simulink model "Wind_PMSG_Transient_R3"  (R2026a)
settings: Solver=ode15s  StopTime=Base.Simulation.StopTime  MaxStep=Base.Simulation.MaxStep
InitFcn:
  | root=fileparts(fileparts(get_param(bdroot,'FileName'))); run(fullfile(root,'parameters','init_wind_pmsg_transient_r3.m'));
undefined symbols (not defined in the file): Base, Control, Converter, Drive, Filter, Grid, PMSG, Wind
libraries: nesl_utility x14, ee_lib x12, fl_lib x4, simulink x2
(part 1 of 2)
Description:
  | Derived transient model: two-mass direct-drive shaft, explicit PMSG dq states and average MSC FOC feeding the accepted switching GSC and grid interface.
settings Model: Creator=fakebob2004  LastModifiedBy=fakebob2004

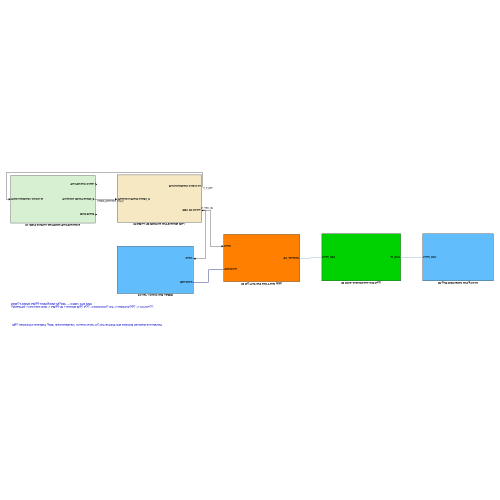
[thumbnail: Simulink's stored preview of the top-level diagram]
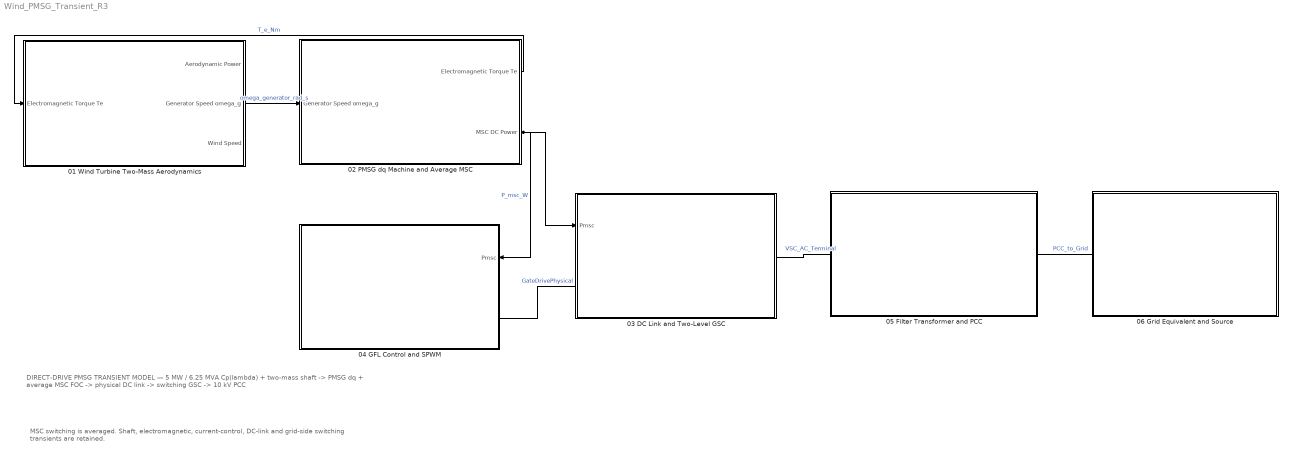
== system Wind_PMSG_Transient_R3 ==
  note: DIRECT-DRIVE PMSG TRANSIENT MODEL — 5 MW / 6.25 MVA
      | Cp(lambda) + two-mass shaft -> PMSG dq + average MSC FOC -> physical DC link -> switching GSC -> 10 kV PCC
  note: MSC switching is averaged. Shaft, electromagnetic, current-control, DC-link and grid-side switching transients are retained.
  01 Wind Turbine Two-Mass Aerodynamics : Subsystem
  02 PMSG dq Machine and Average MSC : Subsystem
  03 DC Link and Two-Level GSC : Subsystem
  04 GFL Control and SPWM : Subsystem
      settings: PortSchema="{\"entries\":[{\"content\":{\"sides\":[{\"content\":{},\"type\":\"ConnectorPlacement.EquallySpacedRectSide\",\"uuid\":\"96295b0e-7f92-4eb5-94fb-1e379a07647e\"},{\"content\":{\"connectorIds\":[\"In1\",\"RConn1\"],\"side\":\"RIGHT\"},\"type\":\"ConnectorPlacement.EquallySpacedRectSide\",\"uuid\":\"831b7b8f-9668-4ddf-9feb-732f61fa57d8\"},{\"content\":{\"side\":\"TOP\"},\"type\":\"ConnectorPlacement.EquallySpacedRectSide\",\"uuid\":\"f19125e2-22e2-45e6-ab3f-ff5603225915\"},{\"content\":{\"side\":\"BOTTOM\"},\"type\":\"ConnectorPlacement.EquallySpacedRectSide\",\"uuid\":\"5342ef29-4f2f-4bd8-ad29-4f76b3f65d35\"}]},\"type\":\"ConnectorPlacement.EquallySpacedConnector\",\"uuid\":\"9af9a57b-5404-446b-bd5e-01cd06fadf4a\"}],\"packageUris\":[\"http://schema.mathworks.com/mf0/Connector/R2020b\"],\"version\":\"1.0\"}"
  05 Filter Transformer and PCC : Subsystem
  06 Grid Equivalent and Source : Subsystem
  wires:
  01 Wind Turbine Two-Mass Aerodynamics/2(Generator Speed omega_g) -> 02 PMSG dq Machine and Average MSC/1(Generator Speed omega_g)  "omega_generator_rad_s"
  02 PMSG dq Machine and Average MSC/1(Electromagnetic Torque Te) -> 01 Wind Turbine Two-Mass Aerodynamics/1(Electromagnetic Torque Te)  "T_e_Nm"
  02 PMSG dq Machine and Average MSC/2(MSC DC Power) -> 03 DC Link and Two-Level GSC/1(Pmsc), 04 GFL Control and SPWM/1(Pmsc)  "P_msc_W"
  connections:
  03 DC Link and Two-Level GSC/RConn1 -- 05 Filter Transformer and PCC/LConn1  "VSC_AC_Terminal"
  05 Filter Transformer and PCC/RConn1 -- 06 Grid Equivalent and Source/LConn1  "PCC_to_Grid"
  04 GFL Control and SPWM/RConn1 -- 03 DC Link and Two-Level GSC/LConn1  "GateDrivePhysical"

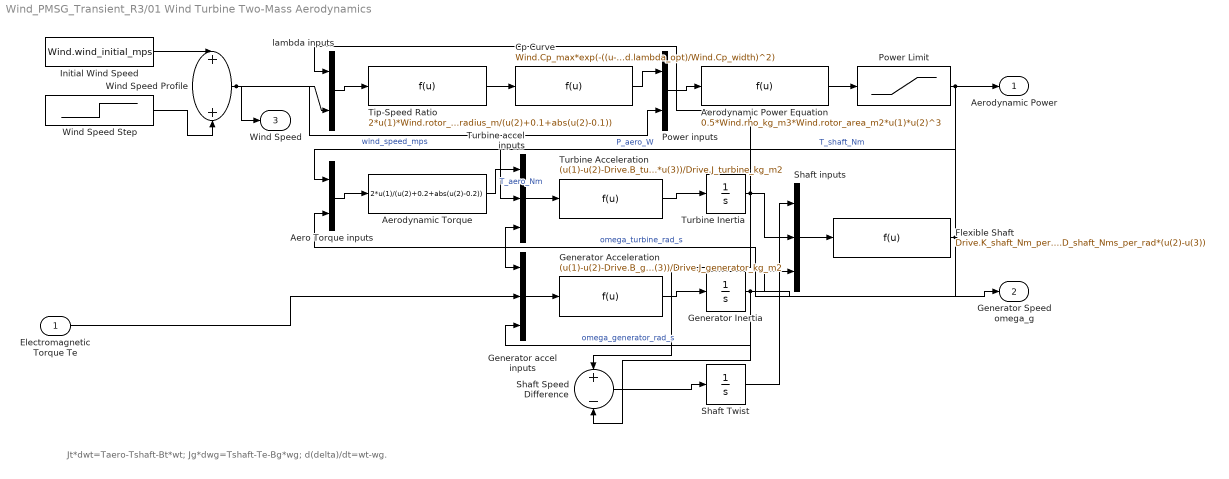
== system Wind_PMSG_Transient_R3/01 Wind Turbine Two-Mass Aerodynamics ==
  note: Jt*dwt=Taero-Tshaft-Bt*wt; Jg*dwg=Tshaft-Te-Bg*wg; d(delta)/dt=wt-wg.
  Electromagnetic Torque Te : Inport
  Aero Torque inputs : Mux  Inputs=2
  Aerodynamic Power Equation : Fcn  Expr=0.5*Wind.rho_kg_m3*Wind.rotor_area_m2*u(1)*u(2)^3
  Aerodynamic Torque : Fcn  Expr=2*u(1)/(u(2)+0.2+abs(u(2)-0.2))
  Cp Curve : Fcn  Expr=Wind.Cp_max*exp(-((u-Wind.lambda_opt)/Wind.Cp_width)^2)
  Flexible Shaft : Fcn  Expr=Drive.K_shaft_Nm_per_rad*u(1)+Drive.D_shaft_Nms_per_rad*(u(2)-u(3))
  Generator Acceleration : Fcn  Expr=(u(1)-u(2)-Drive.B_generator_Nms_per_rad*u(3))/Drive.J_generator_kg_m2
  Generator Inertia : Integrator  InitialCondition=PMSG.Init.omega_rad_s
  Generator accel inputs : Mux  Inputs=3
  Initial Wind Speed : Constant  Value=Wind.wind_initial_mps
  Power Limit : Saturate  UpperLimit=1.10*Wind.P_rated_W  LowerLimit=0
  Power inputs : Mux  Inputs=2
  Shaft Speed Difference : Sum  Inputs=+-
  Shaft Twist : Integrator  InitialCondition=PMSG.Init.shaft_angle_rad
  Shaft inputs : Mux  Inputs=3
  Tip-Speed Ratio : Fcn  Expr=2*u(1)*Wind.rotor_radius_m/(u(2)+0.1+abs(u(2)-0.1))
  Turbine Acceleration : Fcn  Expr=(u(1)-u(2)-Drive.B_turbine_Nms_per_rad*u(3))/Drive.J_turbine_kg_m2
  Turbine Inertia : Integrator  InitialCondition=PMSG.Init.omega_rad_s
  Turbine accel inputs : Mux  Inputs=3
  Wind Speed Profile : Sum
  Wind Speed Step : Step  Time=Wind.wind_step_time_s  FinalValue=Wind.wind_step_mps  SampleTime=0
  lambda inputs : Mux  Inputs=2
  Aerodynamic Power : Outport
  Generator Speed omega_g : Outport  Port=2
  Wind Speed : Outport  Port=3
  wires:
  Initial Wind Speed/1 -> Wind Speed Profile/1
  Wind Speed Step/1 -> Wind Speed Profile/2
  Wind Speed Profile/1 -> Wind Speed/1, lambda inputs/2, Power inputs/2  "wind_speed_mps"
  Turbine Inertia/1 -> lambda inputs/1, Aero Torque inputs/2, Turbine accel inputs/3, Shaft Speed Difference/1, Shaft inputs/2  "omega_turbine_rad_s"
  lambda inputs/1 -> Tip-Speed Ratio/1
  Tip-Speed Ratio/1 -> Cp Curve/1
  Cp Curve/1 -> Power inputs/1
  Power inputs/1 -> Aerodynamic Power Equation/1
  Aerodynamic Power Equation/1 -> Power Limit/1
  Power Limit/1 -> Aerodynamic Power/1, Aero Torque inputs/1  "P_aero_W"
  Aero Torque inputs/1 -> Aerodynamic Torque/1
  Aerodynamic Torque/1 -> Turbine accel inputs/1  "T_aero_Nm"
  Flexible Shaft/1 -> Turbine accel inputs/2, Generator accel inputs/1  "T_shaft_Nm"
  Turbine accel inputs/1 -> Turbine Acceleration/1
  Turbine Acceleration/1 -> Turbine Inertia/1
  Electromagnetic Torque Te/1 -> Generator accel inputs/2
  Generator Inertia/1 -> Generator accel inputs/3, Shaft Speed Difference/2, Shaft inputs/3, Generator Speed omega_g/1  "omega_generator_rad_s"
  Generator accel inputs/1 -> Generator Acceleration/1
  Generator Acceleration/1 -> Generator Inertia/1
  Shaft Speed Difference/1 -> Shaft Twist/1
  Shaft Twist/1 -> Shaft inputs/1
  Shaft inputs/1 -> Flexible Shaft/1

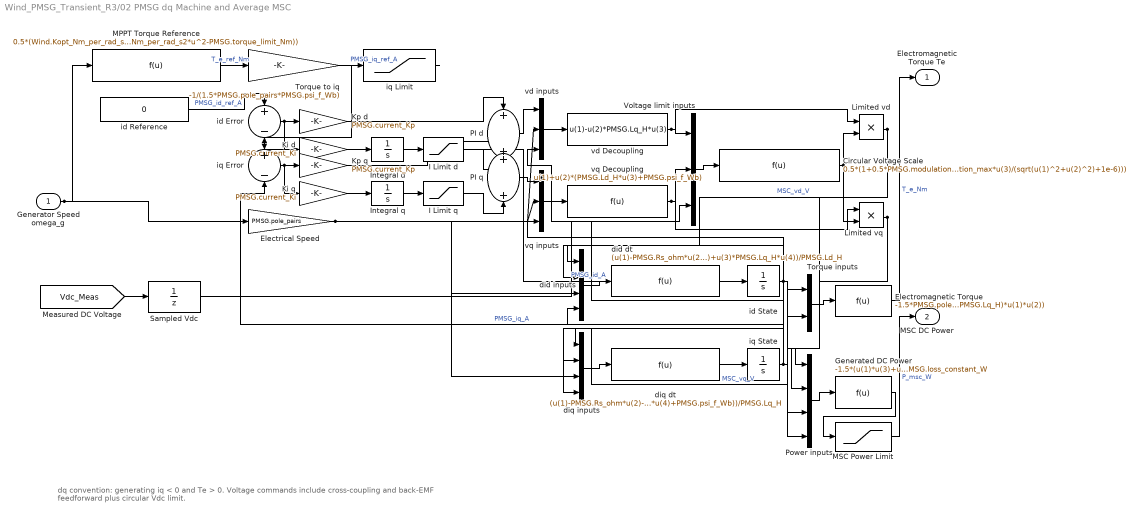
== system Wind_PMSG_Transient_R3/02 PMSG dq Machine and Average MSC ==
  note: dq convention: generating iq < 0 and Te > 0. Voltage commands include cross-coupling and back-EMF feedforward plus circular Vdc limit.
  Generator Speed omega_g : Inport
  Circular Voltage Scale : Fcn  Expr=0.5*(1+0.5*PMSG.modulation_max*u(3)/(sqrt(u(1)^2+u(2)^2)+1e-6)-abs(1-0.5*PMSG.modulation_max*u(3)/(sqrt(u(1)^2+u(2)^2)+1e-6)))
  Electrical Speed : Gain  Gain=PMSG.pole_pairs
  Electromagnetic Torque : Fcn  Expr=-1.5*PMSG.pole_pairs*(PMSG.psi_f_Wb*u(2)+(PMSG.Ld_H-PMSG.Lq_H)*u(1)*u(2))
  Generated DC Power : Fcn  Expr=-1.5*(u(1)*u(3)+u(2)*u(4))*PMSG.msc_efficiency-PMSG.loss_constant_W
  I Limit d : Saturate  UpperLimit=PMSG.integrator_limit_V  LowerLimit=-PMSG.integrator_limit_V
  I Limit q : Saturate  UpperLimit=PMSG.integrator_limit_V  LowerLimit=-PMSG.integrator_limit_V
  Integral d : Integrator  InitialCondition=PMSG.Init.vd_pi_V
  Integral q : Integrator  InitialCondition=PMSG.Init.vq_pi_V
  Ki d : Gain  Gain=PMSG.current_Ki
  Ki q : Gain  Gain=PMSG.current_Ki
  Kp d : Gain  Gain=PMSG.current_Kp
  Kp q : Gain  Gain=PMSG.current_Kp
  Limited vd : Product
  Limited vq : Product
  MPPT Torque Reference : Fcn  Expr=0.5*(Wind.Kopt_Nm_per_rad_s2*u^2+PMSG.torque_limit_Nm-abs(Wind.Kopt_Nm_per_rad_s2*u^2-PMSG.torque_limit_Nm))
  MSC Power Limit : Saturate  UpperLimit=PMSG.Sn_W  LowerLimit=0
  PI d : Sum
  PI q : Sum
  Power inputs : Mux
  Sampled Vdc : UnitDelay  InitialCondition=Converter.Vdc_nom  SampleTime=Control.Ts
  Torque inputs : Mux  Inputs=2
  Torque to iq : Gain  Gain=-1/(1.5*PMSG.pole_pairs*PMSG.psi_f_Wb)
  Voltage limit inputs : Mux  Inputs=3
  did dt : Fcn  Expr=(u(1)-PMSG.Rs_ohm*u(2)+u(3)*PMSG.Lq_H*u(4))/PMSG.Ld_H
  did inputs : Mux
  diq dt : Fcn  Expr=(u(1)-PMSG.Rs_ohm*u(2)-u(3)*(PMSG.Ld_H*u(4)+PMSG.psi_f_Wb))/PMSG.Lq_H
  diq inputs : Mux
  id Error : Sum  Inputs=+-
  id Reference : Constant  Value=0
  id State : Integrator  InitialCondition=PMSG.Init.id_A
  iq Error : Sum  Inputs=+-
  iq Limit : Saturate  UpperLimit=PMSG.current_limit_A  LowerLimit=-PMSG.current_limit_A
  iq State : Integrator  InitialCondition=PMSG.Init.iq_A
  vd Decoupling : Fcn  Expr=u(1)-u(2)*PMSG.Lq_H*u(3)
  vd inputs : Mux  Inputs=3
  vq Decoupling : Fcn  Expr=u(1)+u(2)*(PMSG.Ld_H*u(3)+PMSG.psi_f_Wb)
  vq inputs : Mux  Inputs=3
  Electromagnetic Torque Te : Outport
  MSC DC Power : Outport  Port=2
  wires:
  Generator Speed omega_g/1 -> MPPT Torque Reference/1, Electrical Speed/1
  MPPT Torque Reference/1 -> Torque to iq/1  "T_e_ref_Nm"
  Torque to iq/1 -> iq Limit/1
  iq Limit/1 -> iq Error/1  "PMSG_iq_ref_A"
  id Reference/1 -> id Error/1  "PMSG_id_ref_A"
  id State/1 -> id Error/2, vq inputs/3, did inputs/2, diq inputs/4, Torque inputs/1, Power inputs/3  "PMSG_id_A"
  iq State/1 -> iq Error/2, vd inputs/3, did inputs/4, diq inputs/2, Torque inputs/2, Power inputs/4  "PMSG_iq_A"
  id Error/1 -> Kp d/1, Ki d/1
  Ki d/1 -> Integral d/1
  Integral d/1 -> I Limit d/1
  Kp d/1 -> PI d/1
  I Limit d/1 -> PI d/2
  iq Error/1 -> Kp q/1, Ki q/1
  Ki q/1 -> Integral q/1
  Integral q/1 -> I Limit q/1
  Kp q/1 -> PI q/1
  I Limit q/1 -> PI q/2
  PI d/1 -> vd inputs/1
  Electrical Speed/1 -> vd inputs/2, vq inputs/2, did inputs/3, diq inputs/3
  vd inputs/1 -> vd Decoupling/1
  PI q/1 -> vq inputs/1
  vq inputs/1 -> vq Decoupling/1
  vd Decoupling/1 -> Voltage limit inputs/1, Limited vd/1
  vq Decoupling/1 -> Voltage limit inputs/2, Limited vq/1
  [Vdc_Meas] -> Sampled Vdc/1
  Sampled Vdc/1 -> Voltage limit inputs/3
  Voltage limit inputs/1 -> Circular Voltage Scale/1
  Circular Voltage Scale/1 -> Limited vd/2, Limited vq/2
  Limited vd/1 -> did inputs/1, Power inputs/1  "MSC_vd_V"
  did inputs/1 -> did dt/1
  did dt/1 -> id State/1
  Limited vq/1 -> diq inputs/1, Power inputs/2  "MSC_vq_V"
  diq inputs/1 -> diq dt/1
  diq dt/1 -> iq State/1
  Torque inputs/1 -> Electromagnetic Torque/1
  Electromagnetic Torque/1 -> Electromagnetic Torque Te/1  "T_e_Nm"
  Power inputs/1 -> Generated DC Power/1
  Generated DC Power/1 -> MSC Power Limit/1
  MSC Power Limit/1 -> MSC DC Power/1  "P_msc_W"

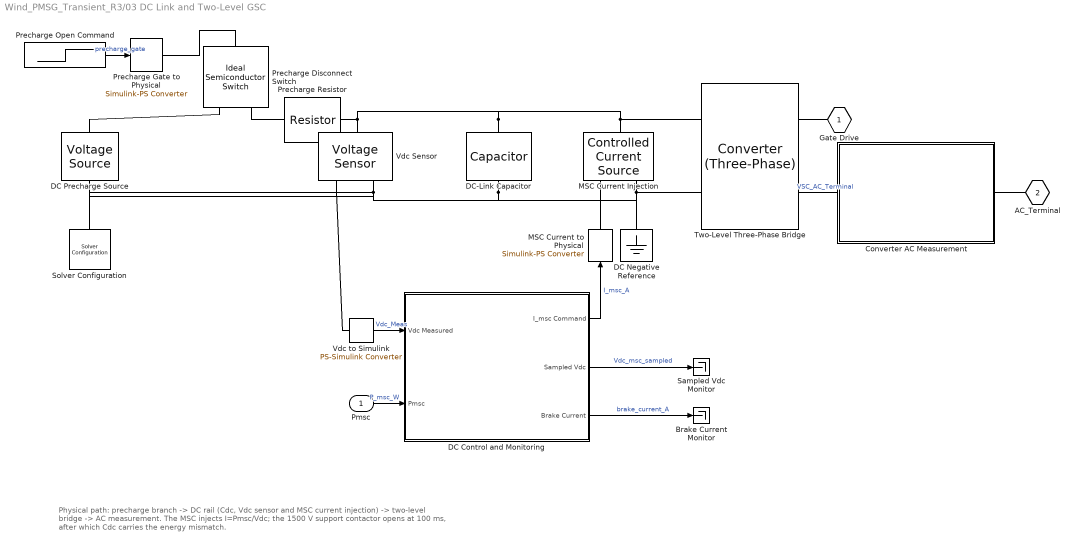
== system Wind_PMSG_Transient_R3/03 DC Link and Two-Level GSC ==
  note: Physical path: precharge branch -> DC rail (Cdc, Vdc sensor and MSC current injection) -> two-level bridge -> AC measurement.
      | The MSC injects I=Pmsc/Vdc; the 1500 V support contactor opens at 100 ms, after which Cdc carries the energy mismatch.
  Pmsc : Inport
  Brake Current Monitor : Terminator
  Converter AC Measurement : Subsystem
  DC Control and Monitoring : Subsystem
  DC Negative Reference : fl_lib/Electrical/Electrical Elements/Electrical Reference
  DC Precharge Source : ee_lib/Sources/Voltage Source  dc_voltage=Converter.Vdc_nom V  ac_voltage=0 V  ac_shift=0 rad  ac_frequency=60 Hz  noise_mode=ee.enum.sources.noise.Disabled  PSD=0 V^2/Hz  sample_time=1e-3 s  repeatability=ee.enum.sources.repeatability.NotRepeatable  user_seed=0  auto_seed=3499211588  i_specify=off  i_priority=None  i=0 A  i_nominal_specify=off  i_nominal_value=1  i_nominal_unit=A  v_specify=off  v_priority=None  v=0 V  v_nominal_specify=off  v_nominal_value=1  v_nominal_unit=V
  DC-Link Capacitor : ee_lib/Passive/Capacitor  cap_option=ee.enum.passive.capacitor.capOption.const  c=Converter.Cdc F  Cvec=[1e-05, 1e-06] F  Vvec=[0, 10] V  CV_table_symmetry=ee.enum.passive.capacitor.tableSymmetry.yes  f_vec=[1, 10] kHz  DFext_vec=[.8, 1.2]  enable_C_tol=ee.enum.toleranceApplication.none  averaging_period=0 s  C_tol=5  tol_distribution=ee.enum.toleranceDistribution.uniform  nSigma=4  r=Converter.Cdc_esr Ohm  g=0 1/Ohm  enable_operating_limits=ee.enum.enable.no  operating_limit_action=ee.enum.passive.reportOpLim.warn  max_working_voltage_range=[-25, 25] V  power_rating=1 W  maxTemperature=85 degC  thermalEnable=false  thermalMass=1 J/K  i_specify=off  i_priority=None  i=0 A  i_nominal_specify=off  i_nominal_value=1  i_nominal_unit=A  v_specify=on  v_priority=High  v=Converter.Vdc_nom V  v_nominal_specify=off  v_nominal_value=1  v_nominal_unit=V  vc_specify=off  vc_priority=High  vc=0 V  vc_nominal_specify=off  vc_nominal_value=1  vc_nominal_unit=V  T_specify=off  T_priority=None  T=298.15 K  T_nominal_specify=off  T_nominal_value=1  T_nominal_unit=K
  MSC Current Injection : fl_lib/Electrical/Electrical Sources/Controlled Current Source
  MSC Current to Physical : nesl_utility/Simulink-PS Converter  PhysicalDomain=network_engine_domain  SubClassName=ps_input  LeftPortType=input  RightPortType=output  PseudoPeriodic=off  Frequencies=[]  NoiseDistribution=none  NoiseParameters=[]  Unit=A  AffineConversion=off  FilteringAndDerivatives=provide  SimscapeFilterOrder=1  InputFilterTimeConstant=0.001  UdotUserProvided=0
  Precharge Disconnect Switch : ee_lib/Semiconductors & Converters/Ideal Semiconductor Switch  port_option=ee.enum.controlport.ps  Ron=Wind.brake_switch_Ron_ohm Ohm  Goff=Wind.brake_switch_Goff_S 1/Ohm  Vth=0.5 V  diode_param=ee.enum.semiconductors.protectionDiode.external  diode_Vf=0.8 V  diode_Ron=0.001 Ohm  diode_Goff=1e-5 1/Ohm  diode_C=50e-9 F  diode_iRM=-235 A  diode_iF=300 A  diode_idot=-50 A/us  diode_trr_param=ee.enum.converters.diodetrr.trr_factor  diode_trr_factor=3  diode_trr=15 us  diode_Qrr=1500 s*uA
  Precharge Gate to Physical : nesl_utility/Simulink-PS Converter  PhysicalDomain=network_engine_domain  SubClassName=ps_input  LeftPortType=input  RightPortType=output  PseudoPeriodic=off  Frequencies=[]  NoiseDistribution=none  NoiseParameters=[]  Unit=1  AffineConversion=off  FilteringAndDerivatives=provide  SimscapeFilterOrder=1  InputFilterTimeConstant=0.001  UdotUserProvided=0
  Precharge Open Command : Step  Time=Wind.precharge_open_time_s  InitialValue=1  FinalValue=0  SampleTime=0
  Precharge Resistor : ee_lib/Passive/Resistor  R=Wind.precharge_R_ohm Ohm  enable_R_tol=ee.enum.toleranceApplication.none  R_tol=5  tol_distribution=ee.enum.toleranceDistribution.uniform  nSigma=4  enable_operating_limits=ee.enum.enable.no  operating_limit_action=ee.enum.passive.reportOpLim.warn  power_rating=1 W  max_working_voltage=100 V  noise_mode=ee.enum.sources.noise.Disabled  Tdevice=25 degC  sample_time=1e-3 s  repeatability=ee.enum.ic.repeatability.notRepeatable  user_seed=0  auto_seed=3890346746  power_derating_T1=70 degC  power_derating_T2=155 degC  operating_temperature_range_vec=[-50, 150] degC  alpha=3.93e-3 1/K  Tmeas=25 degC  thermal_mass=100 J/K  temperature_specify=off  temperature_priority=High  temperature=298.15 K  temperature_nominal_specify=off  temperature_nominal_value=1  temperature_nominal_unit=K
  Sampled Vdc Monitor : Terminator
  Solver Configuration : nesl_utility/Solver Configuration  PhysicalDomain=network_engine_domain  SubClassName=solver  LeftPortType=input  RightPortType=generic  Tones=[]  Harmonics=[]  SimulateNoise=off  Profile=off  UseLocalSampling=off  EnableSwitchedLinearOptims=on  FrequencyDomain=off  UseCCode=off  RelTol=0.001  AbsTol=0.001  MinStep=1e-09  ToWorkspace=off  RevertToSquareIcSolve=off  NumHomotopyIterations=100  PhasorMode=off  PhasorModeNumHarmonics=1  ConsistencySolver=NEWTON_XTOL_AFTER_FTOL  CanonicalOrdering=CANONICAL  OptimizeIntermediates=OPTIMIZED  IndexReductionMethod=DerivativeReplacement  DoDC=off  ResidualTolerance=1e-09  ConsistencyTolSource=GLOBAL  ConsistencyAbsTol=0.001  ConsistencyRelTol=0.001  ConsistencyTolFactor=0.001  UseLocalSolver=off  LocalSolverChoice=NE_BACKWARD_EULER_ADVANCER  ResolveIndetEquations=on  FunctionEvalNumThread=1  LocalSolverSampleTime=0.001  DoFixedCost=off  MaxNonlinIter=3  MaxModeIter=2  ComputeImpulses=off  ImpulseIterations=2  LinearAlgebra=auto  LinearAlgebraNumThread=0  EquationFormulation=NE_TIME_EF  DelaysMemoryBudget=1024  AutomaticFiltering=on  FilteringTimeConstant=0.001  PartitionStorageMethod=AS_NEEDED  PartitionMemoryBudget=1024  PartitionMethod=ROBUST  MultibodyUseLocalSolver=off  MultibodyLocalSolverChoice=ODE1  MultibodyLocalSolverSampleTime=0.001
  Two-Level Three-Phase Bridge : ee_lib/Semiconductors & Converters/Converters/Converter (Three-Phase)  port_option=ee.enum.threePhasePort.composite  fidelity_option=ee.enum.converters.fidelity.detailed  device_type=ee.enum.converters.switchingdevice.ideal  showThermalPort=false  K=0  Vth=Converter.GateThresholdVoltage V  Vgt=1 V  Vgt_off=-1 V  Ih=1 A  Vf=0.8 V  Ron=Converter.SwitchOnResistance Ohm  Rds=0.001 Ohm  Goff=Converter.OffConductance 1/Ohm  Eon_scalar=22.86e-3 J  Eoff_scalar=17.14e-3 J  Eoff_natural_commutation=10e-3 J  Voff=300 V  Iout_scalar=600 A  onCurrentMeasDelay=0 s  useCurrentFromPreviousCycle=false  useVoltageFromPreviousCycle=false  diode_param=ee.enum.converters.protectiondiode.nodynamics  diode_Vf=0.8 V  diode_Ron=0.001 Ohm  diode_Goff=1e-5 1/Ohm  diode_C=50 nF  diode_iRM=-235 A  diode_iF=300 A  diode_idot=-50 A/us  diode_trr_param=ee.enum.converters.diodetrr.trr_factor  diode_trr_factor=3  diode_trr=15 us  diode_Qrr=1500 s*uA  diode_rec_loss_model=ee.enum.diode.reverseRecoveryModel.fixed  diode_ErecVal=0 J  diode_scaleWithIandV=false  diode_ErecMat=zeros(2, 3) J  diode_TjrecVec=[298.15, 398.15] K  diode_IfrecVec=[.1, 1, 10] A  diode_IrecVal=10 A  diode_VrecVal=10 V  diode_tFilter=1 / 1000 / 100 s  thermal_network_parameterization=ee.enum.thermalNetworkTopology.external  Rth=[.08, .5] K/W  Rth_Cauer=[.08, .1, .5] K/W  Rth_Foster=[.08, .14, .22, .16] K/W  thermal_mass_parameterization=ee.enum.thermalNetwork.timeconstant  thermal_mass=[.01, .5] J/K  thermal_mass_Cauer=[.01, .1, .5] J/K  thermal_mass_Foster=[.001, .005, .05, .5] J/K  thermal_time_constant=[.001, .2] s  thermal_time_constant_Cauer=[.001, .1, .2] s  thermal_time_constant_Foster=[7e-05, .0007, .01, .08] s  thermal_mass_initial_temperatures=[25, 25] degC  thermal_mass_initial_temperatures_Cauer=[25, 25, 25] degC  junction_thermal_mass=0.01 J/K  Tvec_initial_Foster=[25, 25, 25, 25] degC  snubber_type=ee.enum.converters.snubber.exclude  Cs=1e-7 F  Rs=0.1 Ohm  Vce_loss=[0, 150, 300] V
  Vdc Sensor : fl_lib/Electrical/Electrical Sensors/Voltage Sensor
  Vdc to Simulink : nesl_utility/PS-Simulink Converter  PhysicalDomain=network_engine_domain  SubClassName=ps_output  LeftPortType=input  RightPortType=output  PseudoPeriodic=off  Frequencies=[]  VectorFormat=inherit  Unit=V  AffineConversion=off
  Gate Drive : PMIOPort  Side=Left
  AC_Terminal : PMIOPort  Port=2  Side=Right
  wires:
  Vdc to Simulink/1 -> DC Control and Monitoring/1(Vdc Measured)  "Vdc_Meas"
  Pmsc/1 -> DC Control and Monitoring/2(Pmsc)  "P_msc_W"
  DC Control and Monitoring/1(I_msc Command) -> MSC Current to Physical/1  "I_msc_A"
  DC Control and Monitoring/2(Sampled Vdc) -> Sampled Vdc Monitor/1  "Vdc_msc_sampled"
  DC Control and Monitoring/3(Brake Current) -> Brake Current Monitor/1  "brake_current_A"
  Precharge Open Command/1 -> Precharge Gate to Physical/1  "precharge_gate"
  connections:
  Gate Drive/RConn1 -- Two-Level Three-Phase Bridge/LConn1
  Vdc Sensor/RConn1 -- Vdc to Simulink/LConn1
  Two-Level Three-Phase Bridge/LConn2 -- Converter AC Measurement/LConn1  "VSC_AC_Terminal"
  Converter AC Measurement/RConn1 -- AC_Terminal/RConn1
  MSC Current to Physical/RConn1 -- MSC Current Injection/RConn1
  DC Precharge Source/LConn1 -- Precharge Disconnect Switch/RConn1
  Precharge Disconnect Switch/RConn2 -- Precharge Resistor/LConn1
  Vdc Sensor/LConn1 -- Precharge Resistor/RConn1 -- DC-Link Capacitor/LConn1 -- MSC Current Injection/LConn1 -- Two-Level Three-Phase Bridge/RConn1
  Vdc Sensor/RConn2 -- DC Precharge Source/RConn1 -- Solver Configuration/RConn1 -- DC-Link Capacitor/RConn1 -- Two-Level Three-Phase Bridge/RConn2 -- MSC Current Injection/RConn2 -- DC Negative Reference/LConn1
  Precharge Gate to Physical/RConn1 -- Precharge Disconnect Switch/LConn1

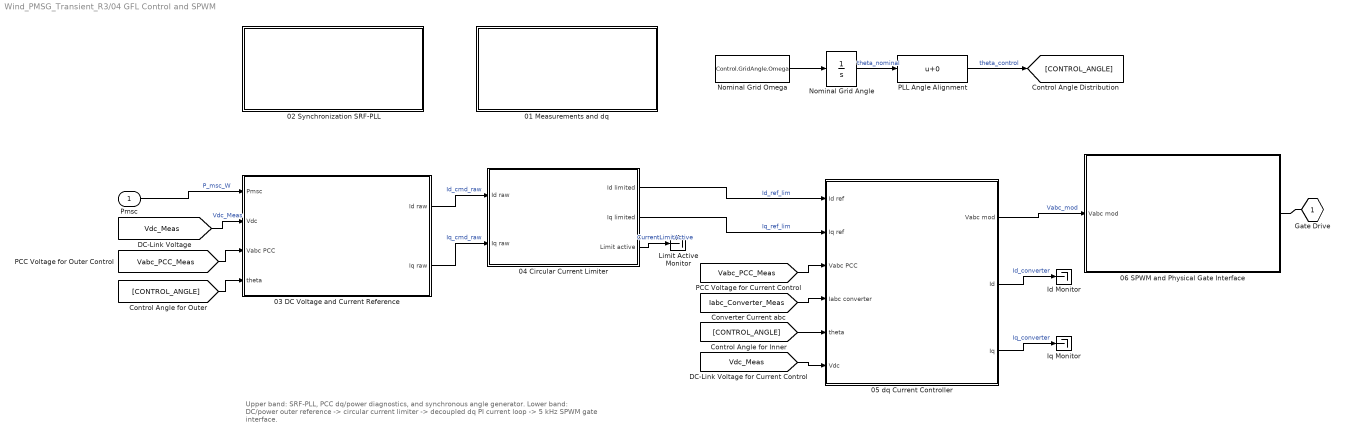
== system Wind_PMSG_Transient_R3/04 GFL Control and SPWM ==
  note: Upper band: SRF-PLL, PCC dq/power diagnostics, and synchronous angle generator. Lower band: DC/power outer reference -> circular current limiter -> decoupled dq PI current loop -> 5 kHz SPWM gate interface.
  Pmsc : Inport
  01 Measurements and dq : Subsystem
  02 Synchronization SRF-PLL : Subsystem
  03 DC Voltage and Current Reference : Subsystem
  04 Circular Current Limiter : Subsystem
  05 dq Current Controller : Subsystem
  06 SPWM and Physical Gate Interface : Subsystem
  Id Monitor : Terminator
  Iq Monitor : Terminator
  Limit Active Monitor : Terminator
  Nominal Grid Angle : Integrator  InitialCondition=Control.GridAngle.Theta0
  Nominal Grid Omega : Constant  Value=Control.GridAngle.Omega
  PLL Angle Alignment : Bias  SaturateOnIntegerOverflow=off
  Gate Drive : PMIOPort  Side=Right
  wires:
  Pmsc/1 -> 03 DC Voltage and Current Reference/1(Pmsc)  "P_msc_W"
  [Vdc_Meas] -> 03 DC Voltage and Current Reference/2(Vdc)  "Vdc_Meas"
  [Vabc_PCC_Meas] -> 03 DC Voltage and Current Reference/3(Vabc PCC)
  Nominal Grid Omega/1 -> Nominal Grid Angle/1
  Nominal Grid Angle/1 -> PLL Angle Alignment/1  "theta_nominal"
  PLL Angle Alignment/1 -> [CONTROL_ANGLE]  "theta_control"
  [CONTROL_ANGLE] -> 03 DC Voltage and Current Reference/4(theta)
  03 DC Voltage and Current Reference/1(Id raw) -> 04 Circular Current Limiter/1(Id raw)  "Id_cmd_raw"
  03 DC Voltage and Current Reference/2(Iq raw) -> 04 Circular Current Limiter/2(Iq raw)  "Iq_cmd_raw"
  04 Circular Current Limiter/1(Id limited) -> 05 dq Current Controller/1(Id ref)  "Id_ref_lim"
  04 Circular Current Limiter/2(Iq limited) -> 05 dq Current Controller/2(Iq ref)  "Iq_ref_lim"
  [Vabc_PCC_Meas] -> 05 dq Current Controller/3(Vabc PCC)
  [Iabc_Converter_Meas] -> 05 dq Current Controller/4(Iabc converter)
  [CONTROL_ANGLE] -> 05 dq Current Controller/5(theta)
  [Vdc_Meas] -> 05 dq Current Controller/6(Vdc)
  05 dq Current Controller/1(Vabc mod) -> 06 SPWM and Physical Gate Interface/1(Vabc mod)  "Vabc_mod"
  05 dq Current Controller/2(Id) -> Id Monitor/1  "Id_converter"
  05 dq Current Controller/3(Iq) -> Iq Monitor/1  "Iq_converter"
  04 Circular Current Limiter/3(Limit active) -> Limit Active Monitor/1  "CurrentLimitActive"
  connections:
  06 SPWM and Physical Gate Interface/RConn1 -- Gate Drive/RConn1

== system Wind_PMSG_Transient_R3/05 Filter Transformer and PCC ==
  note: Direct power path: Rf + Lf -> 0.69/10 kV Y-Y transformer -> PCC VI sensor. Measurements remain internal and logged.
  0.69 kV to 10 kV Step-Up Transformer : ee_lib/Passive/Transformers/Two-Winding Transformer (Three-Phase)  SRated=Transformer.Sn A*V  FRated=Transformer.f Hz  Winding1Connection=ee.enum.windingconnection.Y  VRated1=Transformer.Vll_primary V  Winding2Connection=ee.enum.windingconnection.Y  VRated2=Transformer.Vll_secondary V  CoreType=ee.enum.coretype.threelimb  pu_Rw1=Transformer.R1_pu  pu_Rw2=Transformer.R2_pu  leakage_reactance_option=ee.enum.transformer_leakage.exclude  pu_Xl1=Transformer.X1_pu  pu_Xl2=Transformer.X2_pu  magnetizing_resistance_option=ee.enum.transformer_magnetizingResistance.exclude  pu_Rm=500  magnetizing_reactance_option=ee.enum.transformer_magnetizingReactance.exclude  saturation_option=ee.enum.transformer_saturation.exclude  pu_Xm=Transformer.Xm_pu  current_data=[0, .002, 1, 2]  magnetic_flux_data=[0, 1.2, 1.5, 1.51]  pu_X0=0.5  i1_specify=off  i1_priority=None  i1=[0, 0, 0] A  i1_nominal_specify=off  i1_nominal_value=1  i1_nominal_unit=A  i2_specify=off  i2_priority=None  i2=[0, 0, 0] A  i2_nominal_specify=off  i2_nominal_value=1  i2_nominal_unit=A  phi_specify=off  phi_priority=None  phi=[0, 0, 0]  phi_nominal_specify=off  phi_nominal_value=1  phi_nominal_unit=1
  AC Filter Rf + Lf : ee_lib/Passive/RLC Assemblies/RLC (Three-Phase)  port_option=ee.enum.threePhasePort.composite  component_structure=ee.enum.rlc.structure.SeriesRL  R=Filter.R Ohm  L=Filter.L H  C=1e-6 F  R_parasitic=0 Ohm  G_parasitic=0 1/Ohm  IL_specify=off  IL_priority=High  IL=[0, 0, 0] A  IL_nominal_specify=off  IL_nominal_value=1  IL_nominal_unit=A  VC_specify=off  VC_priority=High  VC=[0, 0, 0] V  VC_nominal_specify=off  VC_nominal_value=1  VC_nominal_unit=V
  Iabc PCC to Simulink : nesl_utility/PS-Simulink Converter  PhysicalDomain=network_engine_domain  SubClassName=ps_output  LeftPortType=input  RightPortType=output  PseudoPeriodic=off  Frequencies=[]  VectorFormat=inherit  Unit=A  AffineConversion=off
  PCC VI Sensor : ee_lib/Sensors & Transducers/Current and Voltage Sensor (Three-Phase)  port_option=ee.enum.threePhasePort.composite  vMeasurementType=ee.enum.vmeasurement.lg  outputUnit=ee.enum.unit.si  SRated=Base.Sn A*V  VRated=Base.Vll_hv V  I_specify=off  I_priority=None  I=[0, 0, 0] A  I_nominal_specify=off  I_nominal_value=1  I_nominal_unit=A  V_specify=off  V_priority=None  V=[0, 0, 0] V  V_nominal_specify=off  V_nominal_value=1  V_nominal_unit=V
  Vabc PCC to Simulink : nesl_utility/PS-Simulink Converter  PhysicalDomain=network_engine_domain  SubClassName=ps_output  LeftPortType=input  RightPortType=output  PseudoPeriodic=off  Frequencies=[]  VectorFormat=inherit  Unit=V  AffineConversion=off
  From_VSC : PMIOPort  Side=Left
  To_Grid : PMIOPort  Port=2  Side=Right
  tag scope: Iabc_PCC_Meas=global, Vabc_PCC_Meas=global
  wires:
  Vabc PCC to Simulink/1 -> [Vabc_PCC_Meas]  "Vabc_PCC_Meas"
  Iabc PCC to Simulink/1 -> [Iabc_PCC_Meas]  "Iabc_PCC_Meas"
  connections:
  From_VSC/RConn1 -- AC Filter Rf + Lf/LConn1
  AC Filter Rf + Lf/RConn1 -- 0.69 kV to 10 kV Step-Up Transformer/LConn1
  0.69 kV to 10 kV Step-Up Transformer/RConn1 -- PCC VI Sensor/LConn1
  PCC VI Sensor/RConn3 -- To_Grid/RConn1
  PCC VI Sensor/RConn1 -- Vabc PCC to Simulink/LConn1
  PCC VI Sensor/RConn2 -- Iabc PCC to Simulink/LConn1

== system Wind_PMSG_Transient_R3/06 Grid Equivalent and Source ==
  note: Single Thevenin impedance: explicit SCR-based Rg + Lg followed by an ideal grounded-wye source (internal source impedance OFF).
  Grid Equivalent Rg + Lg : ee_lib/Passive/RLC Assemblies/RLC (Three-Phase)  port_option=ee.enum.threePhasePort.composite  component_structure=ee.enum.rlc.structure.SeriesRL  R=Grid.R Ohm  L=Grid.L H  C=1e-6 F  R_parasitic=0 Ohm  G_parasitic=0 1/Ohm  IL_specify=off  IL_priority=High  IL=[0, 0, 0] A  IL_nominal_specify=off  IL_nominal_value=1  IL_nominal_unit=A  VC_specify=off  VC_priority=High  VC=[0, 0, 0] V  VC_nominal_specify=off  VC_nominal_value=1  VC_nominal_unit=V
  Grid Neutral Ground : fl_lib/Electrical/Electrical Elements/Electrical Reference
  Ideal Three-Phase Grid Source : ee_lib/Sources/Voltage Source (Three-Phase)  vline_rms=Grid.Vll V  shift=Grid.phase_deg deg  freq=Grid.f Hz  impedance_option=0  SShortCircuit=1e6 A*V  XR=15  R=0.01 Ohm  L=3.97e-4 H  harmonic_option=0  harmonic_orders=[5, 7, 11, 13]  harmonic_ratios=[.1, .1, .1, .1]  G_parasitic=0 1/Ohm  I_specify=off  I_priority=None  I=[0, 0, 0] A  I_nominal_specify=off  I_nominal_value=1  I_nominal_unit=A
  From_PCC : PMIOPort  Side=Left
  connections:
  From_PCC/RConn1 -- Grid Equivalent Rg + Lg/LConn1
  Grid Equivalent Rg + Lg/RConn1 -- Ideal Three-Phase Grid Source/RConn1
  Ideal Three-Phase Grid Source/LConn1 -- Grid Neutral Ground/LConn1

== system Wind_PMSG_Transient_R3/03 DC Link and Two-Level GSC/Converter AC Measurement ==
  note: VSC-side phase voltage, line voltage, and switching current are measured before the RL filter.
  Converter Terminal VI Sensor : ee_lib/Sensors & Transducers/Current and Voltage Sensor (Three-Phase)  port_option=ee.enum.threePhasePort.composite  vMeasurementType=ee.enum.vmeasurement.lg  outputUnit=ee.enum.unit.si  SRated=Base.Sn A*V  VRated=Base.Vll_lv V  I_specify=off  I_priority=None  I=[0, 0, 0] A  I_nominal_specify=off  I_nominal_value=1  I_nominal_unit=A  V_specify=off  V_priority=None  V=[0, 0, 0] V  V_nominal_specify=off  V_nominal_value=1  V_nominal_unit=V
  Iabc to Simulink : nesl_utility/PS-Simulink Converter  PhysicalDomain=network_engine_domain  SubClassName=ps_output  LeftPortType=input  RightPortType=output  PseudoPeriodic=off  Frequencies=[]  VectorFormat=inherit  Unit=A  AffineConversion=off
  Line Voltage Calculation : Subsystem
  Vabc to Simulink : nesl_utility/PS-Simulink Converter  PhysicalDomain=network_engine_domain  SubClassName=ps_output  LeftPortType=input  RightPortType=output  PseudoPeriodic=off  Frequencies=[]  VectorFormat=inherit  Unit=V  AffineConversion=off
  Vll Internal Monitor : Terminator
  From_VSC : PMIOPort  Side=Left
  To_Filter : PMIOPort  Port=2  Side=Right
  tag scope: Iabc_Converter_Meas=global, Vabc_Converter_Meas=global
  wires:
  Vabc to Simulink/1 -> Line Voltage Calculation/1(Vabc), [Vabc_Converter_Meas]  "Vabc_Converter_Meas"
  Line Voltage Calculation/1(Vll) -> Vll Internal Monitor/1  "Vll_inv"
  Iabc to Simulink/1 -> [Iabc_Converter_Meas]  "Iabc_Converter_Meas"
  connections:
  From_VSC/RConn1 -- Converter Terminal VI Sensor/LConn1
  Converter Terminal VI Sensor/RConn3 -- To_Filter/RConn1
  Converter Terminal VI Sensor/RConn1 -- Vabc to Simulink/LConn1
  Converter Terminal VI Sensor/RConn2 -- Iabc to Simulink/LConn1

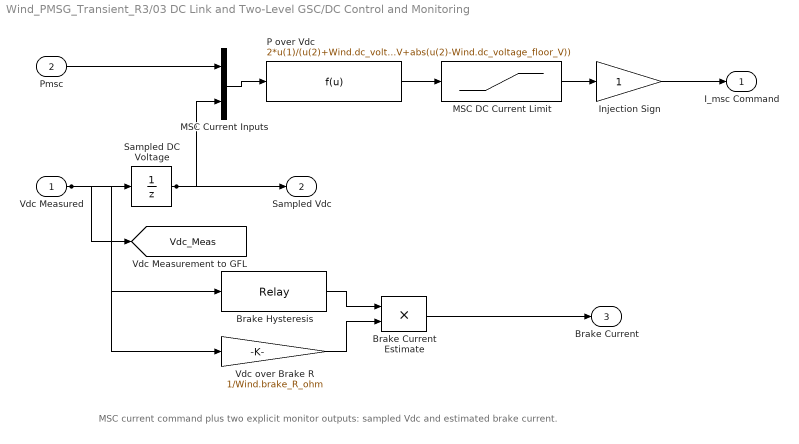
== system Wind_PMSG_Transient_R3/03 DC Link and Two-Level GSC/DC Control and Monitoring ==
  note: MSC current command plus two explicit monitor outputs: sampled Vdc and estimated brake current.
  Vdc Measured : Inport
  Pmsc : Inport  Port=2
  Brake Current Estimate : Product
  Brake Hysteresis : Relay  OnSwitchValue=Wind.brake_on_V  OffSwitchValue=Wind.brake_off_V
  Injection Sign : Gain
  MSC Current Inputs : Mux  Inputs=2
  MSC DC Current Limit : Saturate  UpperLimit=Wind.dc_current_limit_A  LowerLimit=0
  P over Vdc : Fcn  Expr=2*u(1)/(u(2)+Wind.dc_voltage_floor_V+abs(u(2)-Wind.dc_voltage_floor_V))
  Sampled DC Voltage : UnitDelay  InitialCondition=Converter.Vdc_nom  SampleTime=Control.Ts
  Vdc over Brake R : Gain  Gain=1/Wind.brake_R_ohm
  I_msc Command : Outport
  Sampled Vdc : Outport  Port=2
  Brake Current : Outport  Port=3
  tag scope: Vdc_Meas=global
  wires:
  Pmsc/1 -> MSC Current Inputs/1
  Vdc Measured/1 -> Sampled DC Voltage/1, [Vdc_Meas], Brake Hysteresis/1, Vdc over Brake R/1
  Sampled DC Voltage/1 -> MSC Current Inputs/2, Sampled Vdc/1
  MSC Current Inputs/1 -> P over Vdc/1
  P over Vdc/1 -> MSC DC Current Limit/1
  MSC DC Current Limit/1 -> Injection Sign/1
  Injection Sign/1 -> I_msc Command/1
  Brake Hysteresis/1 -> Brake Current Estimate/1
  Vdc over Brake R/1 -> Brake Current Estimate/2
  Brake Current Estimate/1 -> Brake Current/1

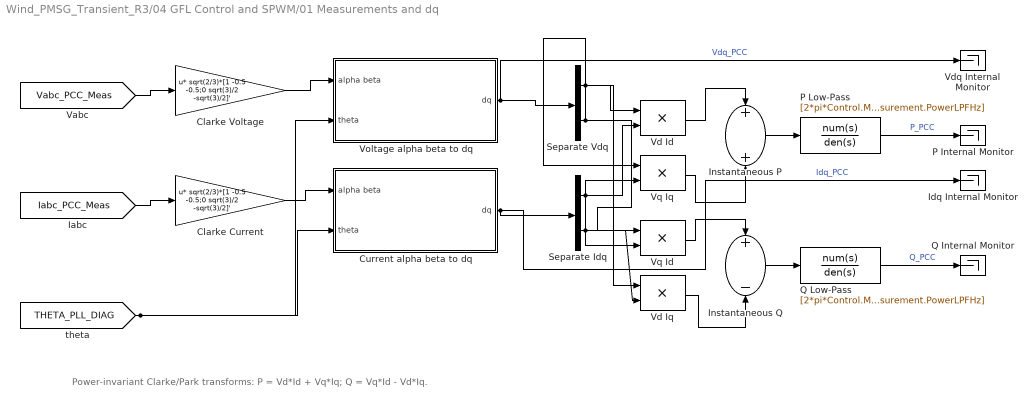
== system Wind_PMSG_Transient_R3/04 GFL Control and SPWM/01 Measurements and dq ==
  note: Power-invariant Clarke/Park transforms: P = Vd*Id + Vq*Iq; Q = Vq*Id - Vd*Iq.
  Clarke Current : Gain  Gain=sqrt(2/3)*[1 -0.5 -0.5;0 sqrt(3)/2 -sqrt(3)/2]'  Multiplication=Matrix(u*K)
  Clarke Voltage : Gain  Gain=sqrt(2/3)*[1 -0.5 -0.5;0 sqrt(3)/2 -sqrt(3)/2]'  Multiplication=Matrix(u*K)
  Current alpha beta to dq : Subsystem
  Idq Internal Monitor : Terminator
  Instantaneous P : Sum
  Instantaneous Q : Sum  Inputs=+-
  P Internal Monitor : Terminator
  P Low-Pass : TransferFcn  Numerator=[2*pi*Control.Measurement.PowerLPFHz]  Denominator=[1 2*pi*Control.Measurement.PowerLPFHz]
  Q Internal Monitor : Terminator
  Q Low-Pass : TransferFcn  Numerator=[2*pi*Control.Measurement.PowerLPFHz]  Denominator=[1 2*pi*Control.Measurement.PowerLPFHz]
  Separate Idq : Demux  Outputs=2
  Separate Vdq : Demux  Outputs=2
  Vd Id : Product
  Vd Iq : Product
  Vdq Internal Monitor : Terminator
  Voltage alpha beta to dq : Subsystem
  Vq Id : Product
  Vq Iq : Product
  wires:
  [Iabc_PCC_Meas] -> Clarke Current/1
  [Vabc_PCC_Meas] -> Clarke Voltage/1
  Clarke Current/1 -> Current alpha beta to dq/1(alpha beta)
  [THETA_PLL_DIAG] -> Current alpha beta to dq/2(theta), Voltage alpha beta to dq/2(theta)
  Current alpha beta to dq/1(dq) -> Idq Internal Monitor/1, Separate Idq/1  "Idq_PCC"
  Vd Id/1 -> Instantaneous P/1
  Vq Iq/1 -> Instantaneous P/2
  Vq Id/1 -> Instantaneous Q/1
  Vd Iq/1 -> Instantaneous Q/2
  P Low-Pass/1 -> P Internal Monitor/1  "P_PCC"
  Instantaneous P/1 -> P Low-Pass/1
  Q Low-Pass/1 -> Q Internal Monitor/1  "Q_PCC"
  Instantaneous Q/1 -> Q Low-Pass/1
  Voltage alpha beta to dq/1(dq) -> Separate Vdq/1, Vdq Internal Monitor/1  "Vdq_PCC"
  Separate Vdq/1 -> Vd Id/1, Vd Iq/1
  Separate Idq/1 -> Vd Id/2, Vq Id/2
  Separate Idq/2 -> Vd Iq/2, Vq Iq/2
  Clarke Voltage/1 -> Voltage alpha beta to dq/1(alpha beta)
  Separate Vdq/2 -> Vq Id/1, Vq Iq/1

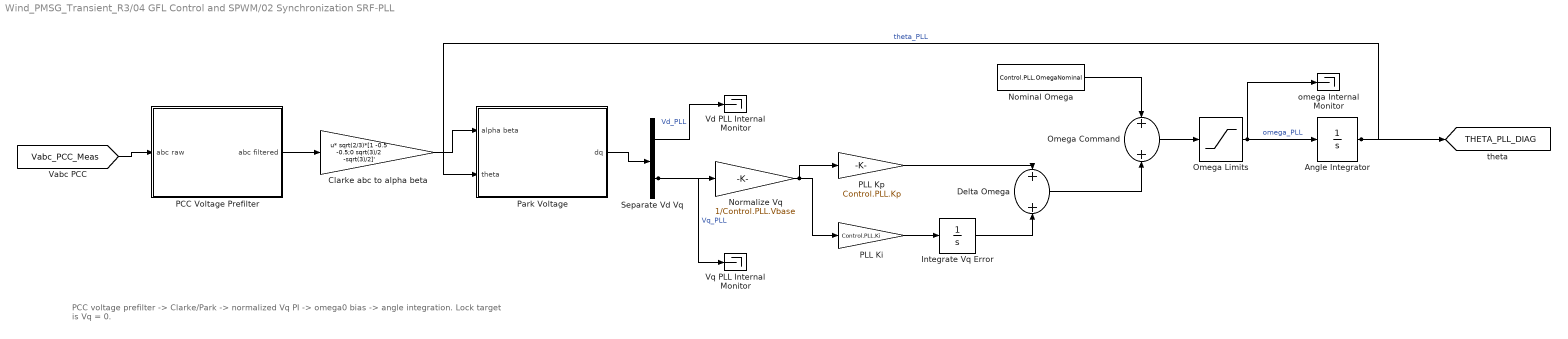
== system Wind_PMSG_Transient_R3/04 GFL Control and SPWM/02 Synchronization SRF-PLL ==
  note: PCC voltage prefilter -> Clarke/Park -> normalized Vq PI -> omega0 bias -> angle integration. Lock target is Vq = 0.
  Angle Integrator : Integrator  InitialCondition=Control.PLL.Theta0
  Clarke abc to alpha beta : Gain  Gain=sqrt(2/3)*[1 -0.5 -0.5;0 sqrt(3)/2 -sqrt(3)/2]'  Multiplication=Matrix(u*K)
  Delta Omega : Sum
  Integrate Vq Error : Integrator
  Nominal Omega : Constant  Value=Control.PLL.OmegaNominal
  Normalize Vq : Gain  Gain=1/Control.PLL.Vbase
  Omega Command : Sum
  Omega Limits : Saturate  UpperLimit=Control.PLL.OmegaMax  LowerLimit=Control.PLL.OmegaMin
  PCC Voltage Prefilter : Subsystem
  PLL Ki : Gain  Gain=Control.PLL.Ki
  PLL Kp : Gain  Gain=Control.PLL.Kp
  Park Voltage : Subsystem
  Separate Vd Vq : Demux  Outputs=2
  Vd PLL Internal Monitor : Terminator
  Vq PLL Internal Monitor : Terminator
  omega Internal Monitor : Terminator
  tag scope: THETA_PLL_DIAG=global
  wires:
  Omega Limits/1 -> Angle Integrator/1, omega Internal Monitor/1  "omega_PLL"
  PCC Voltage Prefilter/1(abc filtered) -> Clarke abc to alpha beta/1
  PLL Kp/1 -> Delta Omega/1
  Integrate Vq Error/1 -> Delta Omega/2
  PLL Ki/1 -> Integrate Vq Error/1
  Separate Vd Vq/2 -> Normalize Vq/1, Vq PLL Internal Monitor/1  "Vq_PLL"
  Nominal Omega/1 -> Omega Command/1
  Delta Omega/1 -> Omega Command/2
  Omega Command/1 -> Omega Limits/1
  [Vabc_PCC_Meas] -> PCC Voltage Prefilter/1(abc raw)
  Normalize Vq/1 -> PLL Ki/1, PLL Kp/1
  Clarke abc to alpha beta/1 -> Park Voltage/1(alpha beta)
  Angle Integrator/1 -> Park Voltage/2(theta), [THETA_PLL_DIAG]  "theta_PLL"
  Park Voltage/1(dq) -> Separate Vd Vq/1
  Separate Vd Vq/1 -> Vd PLL Internal Monitor/1  "Vd_PLL"

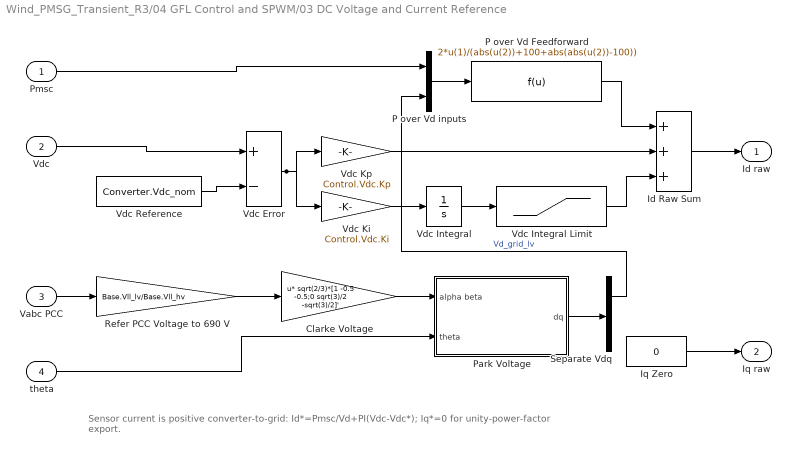
== system Wind_PMSG_Transient_R3/04 GFL Control and SPWM/03 DC Voltage and Current Reference ==
  note: Sensor current is positive converter-to-grid: Id*=Pmsc/Vd+PI(Vdc-Vdc*); Iq*=0 for unity-power-factor export.
  Pmsc : Inport
  Vdc : Inport  Port=2
  Vabc PCC : Inport  Port=3
  theta : Inport  Port=4
  Clarke Voltage : Gain  Gain=sqrt(2/3)*[1 -0.5 -0.5;0 sqrt(3)/2 -sqrt(3)/2]'  Multiplication=Matrix(u*K)
  Id Raw Sum : Sum  Inputs=+++
  Iq Zero : Constant  Value=0
  P over Vd Feedforward : Fcn  Expr=2*u(1)/(abs(u(2))+100+abs(abs(u(2))-100))
  P over Vd inputs : Mux  Inputs=2
  Park Voltage : Subsystem
  Refer PCC Voltage to 690 V : Gain  Gain=Base.Vll_lv/Base.Vll_hv
  Separate Vdq : Demux  Outputs=2
  Vdc Error : Sum  Inputs=+-
  Vdc Integral : Integrator
  Vdc Integral Limit : Saturate  UpperLimit=Control.Vdc.IntegratorLimit  LowerLimit=-Control.Vdc.IntegratorLimit
  Vdc Ki : Gain  Gain=Control.Vdc.Ki
  Vdc Kp : Gain  Gain=Control.Vdc.Kp
  Vdc Reference : Constant  Value=Converter.Vdc_nom
  Id raw : Outport
  Iq raw : Outport  Port=2
  wires:
  Vabc PCC/1 -> Refer PCC Voltage to 690 V/1
  Refer PCC Voltage to 690 V/1 -> Clarke Voltage/1
  Clarke Voltage/1 -> Park Voltage/1(alpha beta)
  theta/1 -> Park Voltage/2(theta)
  Park Voltage/1(dq) -> Separate Vdq/1
  Pmsc/1 -> P over Vd inputs/1
  Separate Vdq/1 -> P over Vd inputs/2  "Vd_grid_lv"
  P over Vd inputs/1 -> P over Vd Feedforward/1
  Vdc/1 -> Vdc Error/1
  Vdc Reference/1 -> Vdc Error/2
  Vdc Error/1 -> Vdc Kp/1, Vdc Ki/1
  Vdc Ki/1 -> Vdc Integral/1
  Vdc Integral/1 -> Vdc Integral Limit/1
  P over Vd Feedforward/1 -> Id Raw Sum/1
  Vdc Kp/1 -> Id Raw Sum/2
  Vdc Integral Limit/1 -> Id Raw Sum/3
  Id Raw Sum/1 -> Id raw/1
  Iq Zero/1 -> Iq raw/1

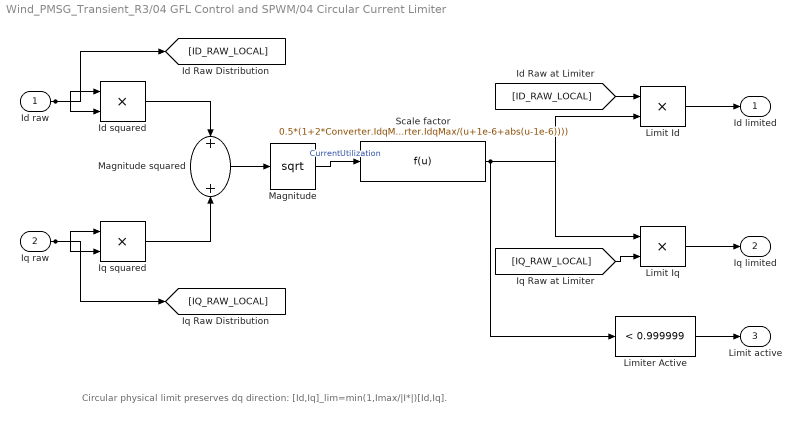
== system Wind_PMSG_Transient_R3/04 GFL Control and SPWM/04 Circular Current Limiter ==
  note: Circular physical limit preserves dq direction: [Id,Iq]_lim=min(1,Imax/|I*|)[Id,Iq].
  Id raw : Inport
  Iq raw : Inport  Port=2
  Id squared : Product
  Iq squared : Product
  Limit Id : Product
  Limit Iq : Product
  Limiter Active : simulink/Logic and Bit Operations/Compare To Constant  relop=<  const=0.999999  OutDataTypeStr=boolean
  Magnitude : Sqrt
  Magnitude squared : Sum
  Scale factor : Fcn  Expr=0.5*(1+2*Converter.IdqMax/(u+1e-6+abs(u-1e-6))-abs(1-2*Converter.IdqMax/(u+1e-6+abs(u-1e-6))))
  Id limited : Outport
  Iq limited : Outport  Port=2
  Limit active : Outport  Port=3
  wires:
  Id raw/1 -> Id squared/1, Id squared/2, [ID_RAW_LOCAL]
  Iq raw/1 -> Iq squared/1, Iq squared/2, [IQ_RAW_LOCAL]
  Id squared/1 -> Magnitude squared/1
  Iq squared/1 -> Magnitude squared/2
  Magnitude squared/1 -> Magnitude/1
  Magnitude/1 -> Scale factor/1  "CurrentUtilization"
  [ID_RAW_LOCAL] -> Limit Id/1
  Scale factor/1 -> Limit Id/2, Limit Iq/1, Limiter Active/1
  [IQ_RAW_LOCAL] -> Limit Iq/2
  Limit Id/1 -> Id limited/1
  Limit Iq/1 -> Iq limited/1
  Limiter Active/1 -> Limit active/1

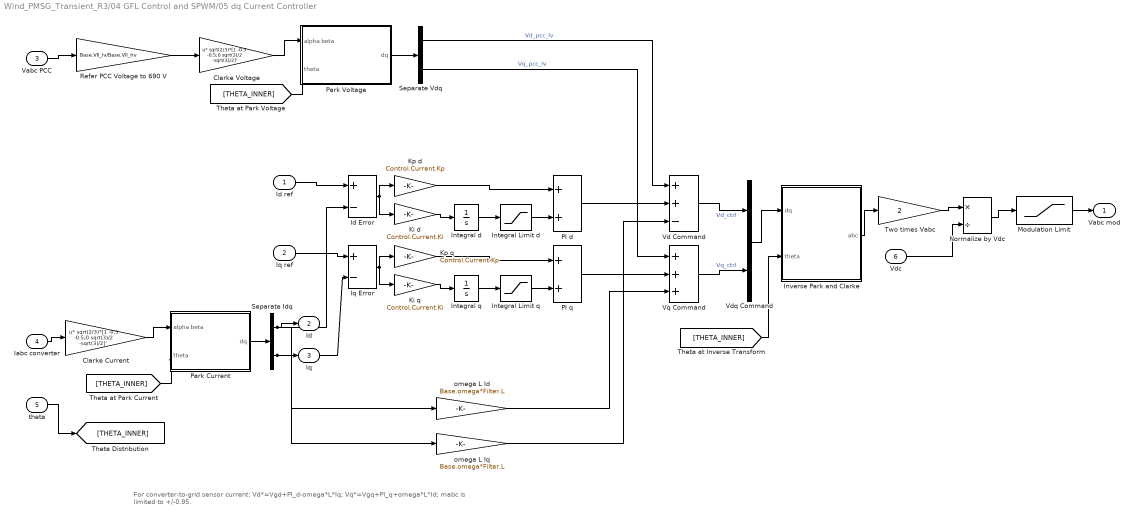
== system Wind_PMSG_Transient_R3/04 GFL Control and SPWM/05 dq Current Controller ==
  note: For converter-to-grid sensor current: Vd*=Vgd+PI_d-omega*L*Iq; Vq*=Vgq+PI_q+omega*L*Id; mabc is limited to +/-0.95.
  Id ref : Inport
  Iq ref : Inport  Port=2
  Vabc PCC : Inport  Port=3
  Iabc converter : Inport  Port=4
  theta : Inport  Port=5
  Vdc : Inport  Port=6
  Clarke Current : Gain  Gain=sqrt(2/3)*[1 -0.5 -0.5;0 sqrt(3)/2 -sqrt(3)/2]'  Multiplication=Matrix(u*K)
  Clarke Voltage : Gain  Gain=sqrt(2/3)*[1 -0.5 -0.5;0 sqrt(3)/2 -sqrt(3)/2]'  Multiplication=Matrix(u*K)
  Id Error : Sum  Inputs=+-
  Integral Limit d : Saturate  UpperLimit=Control.Current.IntegratorLimitV  LowerLimit=-Control.Current.IntegratorLimitV
  Integral Limit q : Saturate  UpperLimit=Control.Current.IntegratorLimitV  LowerLimit=-Control.Current.IntegratorLimitV
  Integral d : Integrator
  Integral q : Integrator
  Inverse Park and Clarke : Subsystem
  Iq Error : Sum  Inputs=+-
  Ki d : Gain  Gain=Control.Current.Ki
  Ki q : Gain  Gain=Control.Current.Ki
  Kp d : Gain  Gain=Control.Current.Kp
  Kp q : Gain  Gain=Control.Current.Kp
  Modulation Limit : Saturate  UpperLimit=Converter.ModulationMax  LowerLimit=-Converter.ModulationMax
  Normalize by Vdc : Product  Inputs=*/
  PI d : Sum
  PI q : Sum
  Park Current : Subsystem
  Park Voltage : Subsystem
  Refer PCC Voltage to 690 V : Gain  Gain=Base.Vll_lv/Base.Vll_hv
  Separate Idq : Demux  Outputs=2
  Separate Vdq : Demux  Outputs=2
  Two times Vabc : Gain  Gain=2
  Vd Command : Sum  Inputs=++-
  Vdq Command : Mux  Inputs=2
  Vq Command : Sum  Inputs=+++
  omega L Id : Gain  Gain=Base.omega*Filter.L
  omega L Iq : Gain  Gain=Base.omega*Filter.L
  Vabc mod : Outport
  Id : Outport  Port=2
  Iq : Outport  Port=3
  wires:
  Vabc PCC/1 -> Refer PCC Voltage to 690 V/1
  Refer PCC Voltage to 690 V/1 -> Clarke Voltage/1
  Clarke Voltage/1 -> Park Voltage/1(alpha beta)
  [THETA_INNER] -> Park Voltage/2(theta)
  Park Voltage/1(dq) -> Separate Vdq/1
  Iabc converter/1 -> Clarke Current/1
  Clarke Current/1 -> Park Current/1(alpha beta)
  [THETA_INNER] -> Park Current/2(theta)
  Park Current/1(dq) -> Separate Idq/1
  Id ref/1 -> Id Error/1
  Separate Idq/1 -> Id Error/2, omega L Id/1, Id/1
  Iq ref/1 -> Iq Error/1
  Separate Idq/2 -> Iq Error/2, omega L Iq/1, Iq/1
  Id Error/1 -> Kp d/1, Ki d/1
  Ki d/1 -> Integral d/1
  Kp d/1 -> PI d/1
  Integral d/1 -> Integral Limit d/1
  Integral Limit d/1 -> PI d/2
  Iq Error/1 -> Kp q/1, Ki q/1
  Ki q/1 -> Integral q/1
  Kp q/1 -> PI q/1
  Integral q/1 -> Integral Limit q/1
  Integral Limit q/1 -> PI q/2
  Separate Vdq/1 -> Vd Command/1  "Vd_pcc_lv"
  PI d/1 -> Vd Command/2
  omega L Iq/1 -> Vd Command/3
  Separate Vdq/2 -> Vq Command/1  "Vq_pcc_lv"
  PI q/1 -> Vq Command/2
  omega L Id/1 -> Vq Command/3
  Vd Command/1 -> Vdq Command/1  "Vd_ctrl"
  Vq Command/1 -> Vdq Command/2  "Vq_ctrl"
  Vdq Command/1 -> Inverse Park and Clarke/1(dq)
  [THETA_INNER] -> Inverse Park and Clarke/2(theta)
  theta/1 -> [THETA_INNER]
  Inverse Park and Clarke/1(abc) -> Two times Vabc/1
  Two times Vabc/1 -> Normalize by Vdc/1
  Vdc/1 -> Normalize by Vdc/2
  Normalize by Vdc/1 -> Modulation Limit/1
  Modulation Limit/1 -> Vabc mod/1

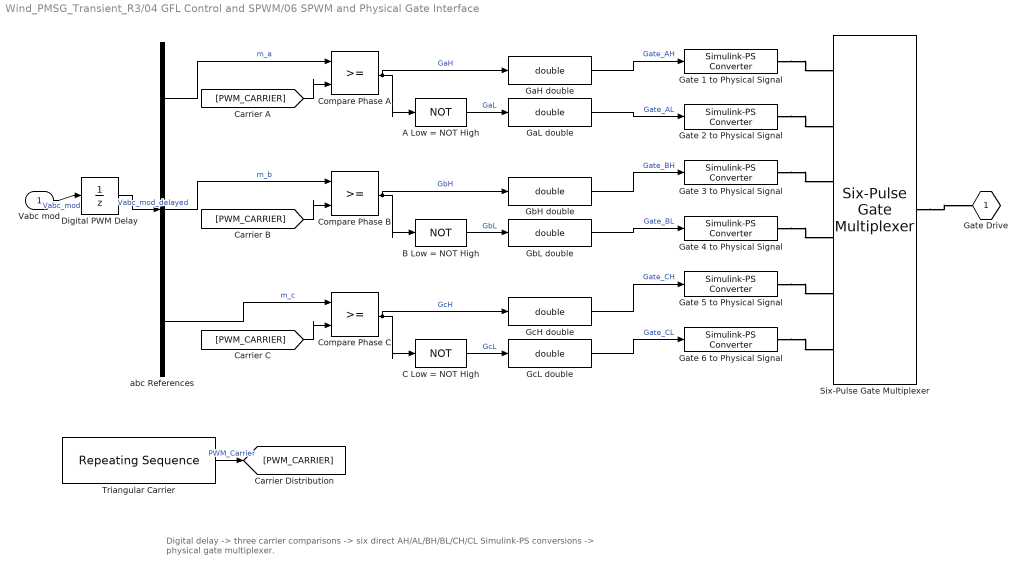
== system Wind_PMSG_Transient_R3/04 GFL Control and SPWM/06 SPWM and Physical Gate Interface ==
  note: Digital delay -> three carrier comparisons -> six direct AH/AL/BH/BL/CH/CL Simulink-PS conversions -> physical gate multiplexer.
  Vabc mod : Inport
  A Low = NOT High : Logic  Operator=NOT  AllPortsSameDT=off  OutDataTypeStr=boolean
  B Low = NOT High : Logic  Operator=NOT  AllPortsSameDT=off  OutDataTypeStr=boolean
  C Low = NOT High : Logic  Operator=NOT  AllPortsSameDT=off  OutDataTypeStr=boolean
  Compare Phase A : RelationalOperator  OutDataTypeStr=boolean  RndMeth=Simplest  InputSameDT=off
  Compare Phase B : RelationalOperator  OutDataTypeStr=boolean  RndMeth=Simplest  InputSameDT=off
  Compare Phase C : RelationalOperator  OutDataTypeStr=boolean  RndMeth=Simplest  InputSameDT=off
  Digital PWM Delay : UnitDelay  InitialCondition=zeros(3,1)  SampleTime=Control.PWM.Ts
  GaH double : DataTypeConversion  OutDataTypeStr=double  SaturateOnIntegerOverflow=off  RndMeth=Floor
  GaL double : DataTypeConversion  OutDataTypeStr=double  SaturateOnIntegerOverflow=off  RndMeth=Floor
  Gate 1 to Physical Signal : nesl_utility/Simulink-PS Converter  PhysicalDomain=network_engine_domain  SubClassName=ps_input  LeftPortType=input  RightPortType=output  PseudoPeriodic=off  Frequencies=[]  NoiseDistribution=none  NoiseParameters=[]  Unit=V  AffineConversion=off  FilteringAndDerivatives=provide  SimscapeFilterOrder=1  InputFilterTimeConstant=0.001  UdotUserProvided=0
  Gate 2 to Physical Signal : nesl_utility/Simulink-PS Converter  PhysicalDomain=network_engine_domain  SubClassName=ps_input  LeftPortType=input  RightPortType=output  PseudoPeriodic=off  Frequencies=[]  NoiseDistribution=none  NoiseParameters=[]  Unit=V  AffineConversion=off  FilteringAndDerivatives=provide  SimscapeFilterOrder=1  InputFilterTimeConstant=0.001  UdotUserProvided=0
  Gate 3 to Physical Signal : nesl_utility/Simulink-PS Converter  PhysicalDomain=network_engine_domain  SubClassName=ps_input  LeftPortType=input  RightPortType=output  PseudoPeriodic=off  Frequencies=[]  NoiseDistribution=none  NoiseParameters=[]  Unit=V  AffineConversion=off  FilteringAndDerivatives=provide  SimscapeFilterOrder=1  InputFilterTimeConstant=0.001  UdotUserProvided=0
  Gate 4 to Physical Signal : nesl_utility/Simulink-PS Converter  PhysicalDomain=network_engine_domain  SubClassName=ps_input  LeftPortType=input  RightPortType=output  PseudoPeriodic=off  Frequencies=[]  NoiseDistribution=none  NoiseParameters=[]  Unit=V  AffineConversion=off  FilteringAndDerivatives=provide  SimscapeFilterOrder=1  InputFilterTimeConstant=0.001  UdotUserProvided=0
  Gate 5 to Physical Signal : nesl_utility/Simulink-PS Converter  PhysicalDomain=network_engine_domain  SubClassName=ps_input  LeftPortType=input  RightPortType=output  PseudoPeriodic=off  Frequencies=[]  NoiseDistribution=none  NoiseParameters=[]  Unit=V  AffineConversion=off  FilteringAndDerivatives=provide  SimscapeFilterOrder=1  InputFilterTimeConstant=0.001  UdotUserProvided=0
  Gate 6 to Physical Signal : nesl_utility/Simulink-PS Converter  PhysicalDomain=network_engine_domain  SubClassName=ps_input  LeftPortType=input  RightPortType=output  PseudoPeriodic=off  Frequencies=[]  NoiseDistribution=none  NoiseParameters=[]  Unit=V  AffineConversion=off  FilteringAndDerivatives=provide  SimscapeFilterOrder=1  InputFilterTimeConstant=0.001  UdotUserProvided=0
  GbH double : DataTypeConversion  OutDataTypeStr=double  SaturateOnIntegerOverflow=off  RndMeth=Floor
  GbL double : DataTypeConversion  OutDataTypeStr=double  SaturateOnIntegerOverflow=off  RndMeth=Floor
  GcH double : DataTypeConversion  OutDataTypeStr=double  SaturateOnIntegerOverflow=off  RndMeth=Floor
  GcL double : DataTypeConversion  OutDataTypeStr=double  SaturateOnIntegerOverflow=off  RndMeth=Floor
  Six-Pulse Gate Multiplexer : ee_lib/Semiconductors & Converters/Converters/Six-Pulse Gate Multiplexer  port_option=ee.enum.controlport.ps
  Triangular Carrier : simulink/Sources/Repeating Sequence  rep_seq_t=[0 Control.PWM.CarrierPeriod/2 Control.PWM.CarrierPeriod]  rep_seq_y=[-1 1 -1]
  abc References : Demux  Outputs=3
  Gate Drive : PMIOPort  Side=Right
  wires:
  Vabc mod/1 -> Digital PWM Delay/1  "Vabc_mod"
  abc References/1 -> Compare Phase A/1  "m_a"
  [PWM_CARRIER] -> Compare Phase A/2
  Compare Phase A/1 -> GaH double/1, A Low = NOT High/1  "GaH"
  A Low = NOT High/1 -> GaL double/1  "GaL"
  abc References/2 -> Compare Phase B/1  "m_b"
  [PWM_CARRIER] -> Compare Phase B/2
  Compare Phase B/1 -> GbH double/1, B Low = NOT High/1  "GbH"
  B Low = NOT High/1 -> GbL double/1  "GbL"
  abc References/3 -> Compare Phase C/1  "m_c"
  [PWM_CARRIER] -> Compare Phase C/2
  Compare Phase C/1 -> GcH double/1, C Low = NOT High/1  "GcH"
  C Low = NOT High/1 -> GcL double/1  "GcL"
  Digital PWM Delay/1 -> abc References/1  "Vabc_mod_delayed"
  Triangular Carrier/1 -> [PWM_CARRIER]  "PWM_Carrier"
  GaH double/1 -> Gate 1 to Physical Signal/1  "Gate_AH"
  GaL double/1 -> Gate 2 to Physical Signal/1  "Gate_AL"
  GbH double/1 -> Gate 3 to Physical Signal/1  "Gate_BH"
  GbL double/1 -> Gate 4 to Physical Signal/1  "Gate_BL"
  GcH double/1 -> Gate 5 to Physical Signal/1  "Gate_CH"
  GcL double/1 -> Gate 6 to Physical Signal/1  "Gate_CL"
  connections:
  Gate 1 to Physical Signal/RConn1 -- Six-Pulse Gate Multiplexer/LConn1
  Gate 2 to Physical Signal/RConn1 -- Six-Pulse Gate Multiplexer/LConn2
  Gate 3 to Physical Signal/RConn1 -- Six-Pulse Gate Multiplexer/LConn3
  Gate 4 to Physical Signal/RConn1 -- Six-Pulse Gate Multiplexer/LConn4
  Gate 5 to Physical Signal/RConn1 -- Six-Pulse Gate Multiplexer/LConn5
  Gate 6 to Physical Signal/RConn1 -- Six-Pulse Gate Multiplexer/LConn6
  Six-Pulse Gate Multiplexer/RConn1 -- Gate Drive/RConn1

== system Wind_PMSG_Transient_R3/03 DC Link and Two-Level GSC/Converter AC Measurement/Line Voltage Calculation ==
  Vabc : Inport
  Separate abc : Demux  Outputs=3
  Vab = Va - Vb : Sum  Inputs=+-
  Vab Vbc Vca : Mux  Inputs=3
  Vbc = Vb - Vc : Sum  Inputs=+-
  Vca = Vc - Va : Sum  Inputs=+-
  Vll : Outport
  wires:
  Vabc/1 -> Separate abc/1
  Separate abc/1 -> Vab = Va - Vb/1, Vca = Vc - Va/2
  Separate abc/2 -> Vab = Va - Vb/2, Vbc = Vb - Vc/1
  Separate abc/3 -> Vbc = Vb - Vc/2, Vca = Vc - Va/1
  Vab = Va - Vb/1 -> Vab Vbc Vca/1
  Vbc = Vb - Vc/1 -> Vab Vbc Vca/2
  Vca = Vc - Va/1 -> Vab Vbc Vca/3
  Vab Vbc Vca/1 -> Vll/1  "Vll_inv"

== system Wind_PMSG_Transient_R3/04 GFL Control and SPWM/01 Measurements and dq/Current alpha beta to dq ==
  alpha beta : Inport
  theta : Inport  Port=2
  Separate alpha beta : Demux  Outputs=2
  alpha cos : Product
  alpha sin : Product
  beta cos : Product
  beta sin : Product
  cos theta : Trigonometry  Operator=cos
  d = alpha cos + beta sin : Sum
  dq vector : Mux  Inputs=2
  q = -alpha sin + beta cos : Sum  Inputs=-+
  sin theta : Trigonometry
  dq : Outport
  wires:
  alpha beta/1 -> Separate alpha beta/1
  theta/1 -> cos theta/1, sin theta/1
  Separate alpha beta/1 -> alpha cos/1, alpha sin/1
  cos theta/1 -> alpha cos/2, beta cos/2
  Separate alpha beta/2 -> beta sin/1, beta cos/1
  sin theta/1 -> beta sin/2, alpha sin/2
  alpha cos/1 -> d = alpha cos + beta sin/1
  beta sin/1 -> d = alpha cos + beta sin/2
  alpha sin/1 -> q = -alpha sin + beta cos/1
  beta cos/1 -> q = -alpha sin + beta cos/2
  d = alpha cos + beta sin/1 -> dq vector/1
  q = -alpha sin + beta cos/1 -> dq vector/2
  dq vector/1 -> dq/1

== system Wind_PMSG_Transient_R3/04 GFL Control and SPWM/01 Measurements and dq/Voltage alpha beta to dq ==
  alpha beta : Inport
  theta : Inport  Port=2
  Separate alpha beta : Demux  Outputs=2
  alpha cos : Product
  alpha sin : Product
  beta cos : Product
  beta sin : Product
  cos theta : Trigonometry  Operator=cos
  d = alpha cos + beta sin : Sum
  dq vector : Mux  Inputs=2
  q = -alpha sin + beta cos : Sum  Inputs=-+
  sin theta : Trigonometry
  dq : Outport
  wires:
  alpha beta/1 -> Separate alpha beta/1
  theta/1 -> cos theta/1, sin theta/1
  Separate alpha beta/1 -> alpha cos/1, alpha sin/1
  cos theta/1 -> alpha cos/2, beta cos/2
  Separate alpha beta/2 -> beta sin/1, beta cos/1
  sin theta/1 -> beta sin/2, alpha sin/2
  alpha cos/1 -> d = alpha cos + beta sin/1
  beta sin/1 -> d = alpha cos + beta sin/2
  alpha sin/1 -> q = -alpha sin + beta cos/1
  beta cos/1 -> q = -alpha sin + beta cos/2
  d = alpha cos + beta sin/1 -> dq vector/1
  q = -alpha sin + beta cos/1 -> dq vector/2
  dq vector/1 -> dq/1

== system Wind_PMSG_Transient_R3/04 GFL Control and SPWM/02 Synchronization SRF-PLL/PCC Voltage Prefilter ==
  abc raw : Inport
  Filtered abc : Mux  Inputs=3
  Phase A LPF : TransferFcn  Numerator=[2*pi*Control.PLL.VoltagePrefilterHz]  Denominator=[1 2*pi*Control.PLL.VoltagePrefilterHz]
  Phase B LPF : TransferFcn  Numerator=[2*pi*Control.PLL.VoltagePrefilterHz]  Denominator=[1 2*pi*Control.PLL.VoltagePrefilterHz]
  Phase C LPF : TransferFcn  Numerator=[2*pi*Control.PLL.VoltagePrefilterHz]  Denominator=[1 2*pi*Control.PLL.VoltagePrefilterHz]
  Separate abc : Demux  Outputs=3
  abc filtered : Outport
  wires:
  Separate abc/1 -> Phase A LPF/1
  Phase A LPF/1 -> Filtered abc/1
  Separate abc/2 -> Phase B LPF/1
  Phase B LPF/1 -> Filtered abc/2
  Separate abc/3 -> Phase C LPF/1
  Phase C LPF/1 -> Filtered abc/3
  abc raw/1 -> Separate abc/1
  Filtered abc/1 -> abc filtered/1
